simulink model "s_b16a4x512f"  (R2016b)
settings: Solver=VariableStepDiscrete  StartTime=0.0  StopTime=1  RelTol=1e-3
undefined symbols (not defined in the file): fft_stages, n_bits_ants, n_bits_xengs
libraries: xbsIndex_r4 x23057, casper_library_misc x150, xbsReplacements_r4 x9, casper_library_delays x8, xps_library x3
(part 15 of 210)

== system s_b16a4x512f/tvg_control ==
  convert1_{1..8,11..18} (16 alike) : DataTypeConversion  OutDataTypeStr=fixdt('ufix1_En0')  LockScale=on
  convert1_10 : DataTypeConversion  OutDataTypeStr=fixdt('ufix2_En0')  LockScale=on
  convert1_9 : DataTypeConversion  OutDataTypeStr=fixdt('ufix2_En0')  LockScale=on
  convert2_{1..8,11..18} (16 alike) : DataTypeConversion  OutDataTypeStr=fixdt('ufix1_En0')  ConvertRealWorld=Stored Integer (SI)  LockScale=on
  convert2_10 : DataTypeConversion  OutDataTypeStr=fixdt('ufix2_En0')  ConvertRealWorld=Stored Integer (SI)  LockScale=on
  convert2_9 : DataTypeConversion  OutDataTypeStr=fixdt('ufix2_En0')  ConvertRealWorld=Stored Integer (SI)  LockScale=on
  gain_1 : Gain  Gain=524288
  gain_10 : Gain  Gain=256
  gain_11 : Gain  Gain=128
  gain_12 : Gain  Gain=64
  gain_13 : Gain  Gain=32
  gain_14 : Gain  Gain=16
  gain_15 : Gain  Gain=8
  gain_16 : Gain  Gain=4
  gain_17 : Gain  Gain=2
  gain_18 : Gain
  gain_2 : Gain  Gain=262144
  gain_3 : Gain  Gain=131072
  gain_4 : Gain  Gain=65536
  gain_5 : Gain  Gain=32768
  gain_6 : Gain  Gain=16384
  gain_7 : Gain  Gain=8192
  gain_8 : Gain  Gain=4096
  gain_9 : Gain  Gain=1024
  io_delay : xbsIndex_r4/Delay  rst=off  infoeditControl=Selection of Reset will increase slice count due to use of real FFs and instead of SRLs  en=off  latency=0  reg_retiming=on  dbl_ovrd=off  block_type=delay
      settings: infoedit=Hardware notes: A delay line is a chain, each link of which is an SRL16 or SRL32 followed by a flip-flop.
  reint{9..10,17..18} (4 alike) : xbsIndex_r4/Reinterpret  force_arith_type=on  arith_type=Unsigned  force_bin_pt=on  bin_pt=0  block_type=reinterpret
  s_b16a4x512f_tvg_control_user_data_out : xbsIndex_r4/Gateway In  gui_display_data_type=Fixed-point  arith_type=Unsigned  n_bits=32  bin_pt=0  preci_type=Single  exp_width=8  frac_width=24  rows=1  columns=1  quantization="Round  (unbiased: +/- Inf)"  overflow=Saturate  period=1  UseAsADC=off  ADCChannel='1'  interface=None  automatic_assignment=on  address_offset=hex2dec('00')  intf_name=''  intf_description=''  default_value=0  timing_constraint=None  locs_specified=off  LOCs={}  io_standard={}  inherit_from_input=off  hdl_port=on  dbl_ovrd=off  block_type=gatewayin
  sim_{1..18} (18 alike) : Constant  Value=0
  sim_add : Sum  Inputs=++++++++++++++++++  OutDataTypeStr=uint32
  slice_preproc_snap_dv_mux : xbsIndex_r4/Slice  nbits=1  boolean_output=on  mode=Lower Bit Location + Width  bit1=0  base1=MSB of Input  bit0=6  base0=LSB of Input  dbl_ovrd=off  block_type=slice
  slice_preproc_snap_stop_mux : xbsIndex_r4/Slice  nbits=1  boolean_output=off  mode=Lower Bit Location + Width  bit1=0  base1=MSB of Input  bit0=1  base0=LSB of Input  dbl_ovrd=off  block_type=slice
  slice_reord_snap_dv_arm : xbsIndex_r4/Slice  nbits=1  boolean_output=on  mode=Lower Bit Location + Width  bit1=0  base1=MSB of Input  bit0=7  base0=LSB of Input  dbl_ovrd=off  block_type=slice
  slice_reord_snap_dv_mux : xbsIndex_r4/Slice  nbits=2  boolean_output=off  mode=Lower Bit Location + Width  bit1=0  base1=MSB of Input  bit0=10  base0=LSB of Input  dbl_ovrd=off  block_type=slice
  slice_snap_hmc_pkt_mux_we_sel : xbsIndex_r4/Slice  nbits=1  boolean_output=off  mode=Lower Bit Location + Width  bit1=0  base1=MSB of Input  bit0=0  base0=LSB of Input  dbl_ovrd=off  block_type=slice
  slice_snap_reord_stop_sel : xbsIndex_r4/Slice  nbits=1  boolean_output=on  mode=Lower Bit Location + Width  bit1=0  base1=MSB of Input  bit0=5  base0=LSB of Input  dbl_ovrd=off  block_type=slice
  slice_vacc_tvg_ctr_en : xbsIndex_r4/Slice  nbits=1  boolean_output=on  mode=Lower Bit Location + Width  bit1=0  base1=MSB of Input  bit0=14  base0=LSB of Input  dbl_ovrd=off  block_type=slice
  slice_vacc_tvg_data_sel : xbsIndex_r4/Slice  nbits=1  boolean_output=on  mode=Lower Bit Location + Width  bit1=0  base1=MSB of Input  bit0=16  base0=LSB of Input  dbl_ovrd=off  block_type=slice
  slice_vacc_tvg_pulse_en : xbsIndex_r4/Slice  nbits=1  boolean_output=on  mode=Lower Bit Location + Width  bit1=0  base1=MSB of Input  bit0=19  base0=LSB of Input  dbl_ovrd=off  block_type=slice
  slice_vacc_tvg_reset : xbsIndex_r4/Slice  nbits=1  boolean_output=on  mode=Lower Bit Location + Width  bit1=0  base1=MSB of Input  bit0=15  base0=LSB of Input  dbl_ovrd=off  block_type=slice
  slice_vacc_tvg_run : xbsIndex_r4/Slice  nbits=1  boolean_output=on  mode=Lower Bit Location + Width  bit1=0  base1=MSB of Input  bit0=12  base0=LSB of Input  dbl_ovrd=off  block_type=slice
  slice_vacc_tvg_sync_sel : xbsIndex_r4/Slice  nbits=1  boolean_output=on  mode=Lower Bit Location + Width  bit1=0  base1=MSB of Input  bit0=18  base0=LSB of Input  dbl_ovrd=off  block_type=slice
  slice_vacc_tvg_valid_sel : xbsIndex_r4/Slice  nbits=1  boolean_output=on  mode=Lower Bit Location + Width  bit1=0  base1=MSB of Input  bit0=17  base0=LSB of Input  dbl_ovrd=off  block_type=slice
  slice_vacc_tvg_vector_en : xbsIndex_r4/Slice  nbits=1  boolean_output=on  mode=Lower Bit Location + Width  bit1=0  base1=MSB of Input  bit0=13  base0=LSB of Input  dbl_ovrd=off  block_type=slice
  slice_xeng_tvg_data_sel : xbsIndex_r4/Slice  nbits=2  boolean_output=off  mode=Lower Bit Location + Width  bit1=0  base1=MSB of Input  bit0=8  base0=LSB of Input  dbl_ovrd=off  block_type=slice
  slice_xeng_tvg_inj_vector : xbsIndex_r4/Slice  nbits=1  boolean_output=on  mode=Lower Bit Location + Width  bit1=0  base1=MSB of Input  bit0=3  base0=LSB of Input  dbl_ovrd=off  block_type=slice
  slice_xeng_tvg_mcnt_sel : xbsIndex_r4/Slice  nbits=1  boolean_output=on  mode=Lower Bit Location + Width  bit1=0  base1=MSB of Input  bit0=2  base0=LSB of Input  dbl_ovrd=off  block_type=slice
  slice_xeng_tvg_val_sel : xbsIndex_r4/Slice  nbits=1  boolean_output=on  mode=Lower Bit Location + Width  bit1=0  base1=MSB of Input  bit0=4  base0=LSB of Input  dbl_ovrd=off  block_type=slice
  in_vacc_tvg_pulse_en : Outport
  in_vacc_tvg_sync_sel : Outport  Port=2
  in_vacc_tvg_valid_sel : Outport  Port=3
  in_vacc_tvg_data_sel : Outport  Port=4
  in_vacc_tvg_reset : Outport  Port=5
  in_vacc_tvg_ctr_en : Outport  Port=6
  in_vacc_tvg_vector_en : Outport  Port=7
  in_vacc_tvg_run : Outport  Port=8
  in_reord_snap_dv_mux : Outport  Port=9
  in_xeng_tvg_data_sel : Outport  Port=10
  in_reord_snap_dv_arm : Outport  Port=11
  in_preproc_snap_dv_mux : Outport  Port=12
  in_snap_reord_stop_sel : Outport  Port=13
  in_xeng_tvg_val_sel : Outport  Port=14
  in_xeng_tvg_inj_vector : Outport  Port=15
  in_xeng_tvg_mcnt_sel : Outport  Port=16
  in_preproc_snap_stop_mux : Outport  Port=17
  in_snap_hmc_pkt_mux_we_sel : Outport  Port=18
  wires:
  s_b16a4x512f_tvg_control_user_data_out/1 -> io_delay/1
  sim_add/1 -> s_b16a4x512f_tvg_control_user_data_out/1
  sim_1/1 -> convert1_1/1
  convert1_1/1 -> convert2_1/1
  convert2_1/1 -> gain_1/1
  gain_1/1 -> sim_add/1
  io_delay/1 -> slice_vacc_tvg_pulse_en/1, slice_vacc_tvg_sync_sel/1, slice_vacc_tvg_valid_sel/1, slice_vacc_tvg_data_sel/1, slice_vacc_tvg_reset/1, slice_vacc_tvg_ctr_en/1, slice_vacc_tvg_vector_en/1, slice_vacc_tvg_run/1, slice_reord_snap_dv_mux/1, slice_xeng_tvg_data_sel/1, slice_reord_snap_dv_arm/1, slice_preproc_snap_dv_mux/1, slice_snap_reord_stop_sel/1, slice_xeng_tvg_val_sel/1, slice_xeng_tvg_inj_vector/1, slice_xeng_tvg_mcnt_sel/1, slice_preproc_snap_stop_mux/1, slice_snap_hmc_pkt_mux_we_sel/1
  slice_vacc_tvg_pulse_en/1 -> in_vacc_tvg_pulse_en/1
  sim_2/1 -> convert1_2/1
  convert1_2/1 -> convert2_2/1
  convert2_2/1 -> gain_2/1
  gain_2/1 -> sim_add/2
  slice_vacc_tvg_sync_sel/1 -> in_vacc_tvg_sync_sel/1
  sim_3/1 -> convert1_3/1
  convert1_3/1 -> convert2_3/1
  convert2_3/1 -> gain_3/1
  gain_3/1 -> sim_add/3
  slice_vacc_tvg_valid_sel/1 -> in_vacc_tvg_valid_sel/1
  sim_4/1 -> convert1_4/1
  convert1_4/1 -> convert2_4/1
  convert2_4/1 -> gain_4/1
  gain_4/1 -> sim_add/4
  slice_vacc_tvg_data_sel/1 -> in_vacc_tvg_data_sel/1
  sim_5/1 -> convert1_5/1
  convert1_5/1 -> convert2_5/1
  convert2_5/1 -> gain_5/1
  gain_5/1 -> sim_add/5
  slice_vacc_tvg_reset/1 -> in_vacc_tvg_reset/1
  sim_6/1 -> convert1_6/1
  convert1_6/1 -> convert2_6/1
  convert2_6/1 -> gain_6/1
  gain_6/1 -> sim_add/6
  slice_vacc_tvg_ctr_en/1 -> in_vacc_tvg_ctr_en/1
  sim_7/1 -> convert1_7/1
  convert1_7/1 -> convert2_7/1
  convert2_7/1 -> gain_7/1
  gain_7/1 -> sim_add/7
  slice_vacc_tvg_vector_en/1 -> in_vacc_tvg_vector_en/1
  sim_8/1 -> convert1_8/1
  convert1_8/1 -> convert2_8/1
  convert2_8/1 -> gain_8/1
  gain_8/1 -> sim_add/8
  slice_vacc_tvg_run/1 -> in_vacc_tvg_run/1
  sim_9/1 -> convert1_9/1
  convert1_9/1 -> convert2_9/1
  convert2_9/1 -> gain_9/1
  gain_9/1 -> sim_add/9
  slice_reord_snap_dv_mux/1 -> reint9/1
  reint9/1 -> in_reord_snap_dv_mux/1
  sim_10/1 -> convert1_10/1
  convert1_10/1 -> convert2_10/1
  convert2_10/1 -> gain_10/1
  gain_10/1 -> sim_add/10
  slice_xeng_tvg_data_sel/1 -> reint10/1
  reint10/1 -> in_xeng_tvg_data_sel/1
  sim_11/1 -> convert1_11/1
  convert1_11/1 -> convert2_11/1
  convert2_11/1 -> gain_11/1
  gain_11/1 -> sim_add/11
  slice_reord_snap_dv_arm/1 -> in_reord_snap_dv_arm/1
  sim_12/1 -> convert1_12/1
  convert1_12/1 -> convert2_12/1
  convert2_12/1 -> gain_12/1
  gain_12/1 -> sim_add/12
  slice_preproc_snap_dv_mux/1 -> in_preproc_snap_dv_mux/1
  sim_13/1 -> convert1_13/1
  convert1_13/1 -> convert2_13/1
  convert2_13/1 -> gain_13/1
  gain_13/1 -> sim_add/13
  slice_snap_reord_stop_sel/1 -> in_snap_reord_stop_sel/1
  sim_14/1 -> convert1_14/1
  convert1_14/1 -> convert2_14/1
  convert2_14/1 -> gain_14/1
  gain_14/1 -> sim_add/14
  slice_xeng_tvg_val_sel/1 -> in_xeng_tvg_val_sel/1
  sim_15/1 -> convert1_15/1
  convert1_15/1 -> convert2_15/1
  convert2_15/1 -> gain_15/1
  gain_15/1 -> sim_add/15
  slice_xeng_tvg_inj_vector/1 -> in_xeng_tvg_inj_vector/1
  sim_16/1 -> convert1_16/1
  convert1_16/1 -> convert2_16/1
  convert2_16/1 -> gain_16/1
  gain_16/1 -> sim_add/16
  slice_xeng_tvg_mcnt_sel/1 -> in_xeng_tvg_mcnt_sel/1
  sim_17/1 -> convert1_17/1
  convert1_17/1 -> convert2_17/1
  convert2_17/1 -> gain_17/1
  gain_17/1 -> sim_add/17
  slice_preproc_snap_stop_mux/1 -> reint17/1
  reint17/1 -> in_preproc_snap_stop_mux/1
  sim_18/1 -> convert1_18/1
  convert1_18/1 -> convert2_18/1
  convert2_18/1 -> gain_18/1
  gain_18/1 -> sim_add/18
  slice_snap_hmc_pkt_mux_we_sel/1 -> reint18/1
  reint18/1 -> in_snap_hmc_pkt_mux_we_sel/1

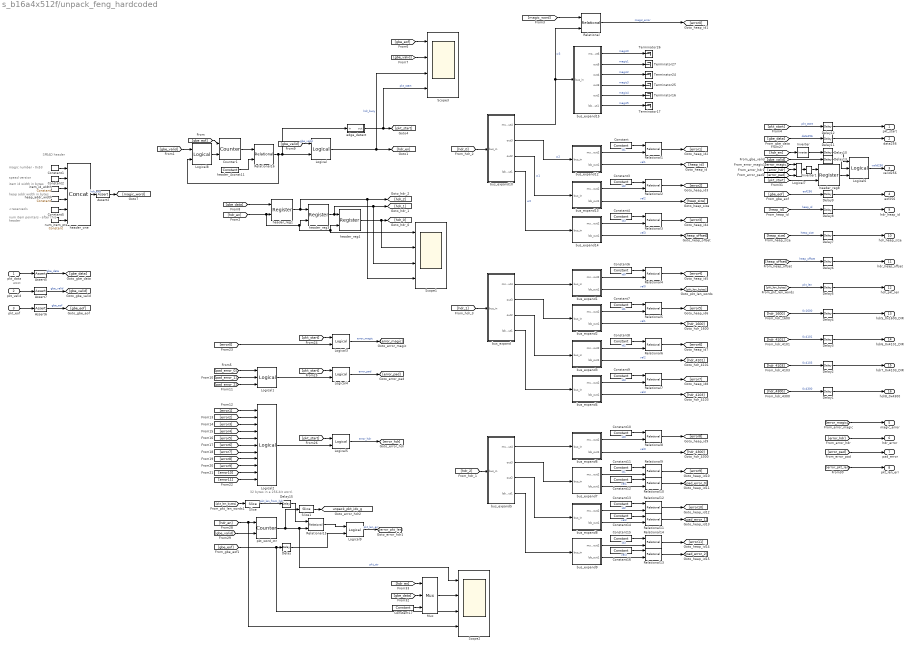
== system s_b16a4x512f/unpack_feng_hardcoded ==
  note: 32 bytes in a 256-bit word.
  note: woot
  note: SPEAD header
  note: magic number - 0x53
  note: spead version
  note: item id width in bytes
  note: heap addr width in bytes
  note: <reserved>
  note: num item pointers -
      | after this header
  pkt_data : Inport
  pkt_valid : Inport  Port=2
  pkt_eof : Inport  Port=3
  Assert2 : xbsIndex_r4/Assert  assert_type=on  type_source=Explicitly  gui_display_data_type=Fixed-point  arith_type=Unsigned  n_bits=64  bin_pt=0  preci_type=Single  exp_width=8  frac_width=24  assert_rate=off  rate_source=Explicitly  period=1  output_port=on  block_type=assert
      settings: block_version=10.1.3
  Assert5 : xbsIndex_r4/Assert  assert_type=on  type_source=Explicitly  gui_display_data_type=Fixed-point  arith_type=Unsigned  n_bits=256  bin_pt=0  preci_type=Single  exp_width=8  frac_width=24  assert_rate=off  rate_source=Explicitly  period=1  output_port=on  block_type=assert
      settings: block_version=10.1.3
  Assert6 : xbsIndex_r4/Assert  assert_type=on  type_source=Explicitly  gui_display_data_type=Boolean  arith_type=Boolean  n_bits=spead_msw  bin_pt=0  preci_type=Single  exp_width=8  frac_width=24  assert_rate=off  rate_source=Explicitly  period=1  output_port=on  block_type=assert
      settings: block_version=10.1.3
  Assert7 : xbsIndex_r4/Assert  assert_type=on  type_source=Explicitly  gui_display_data_type=Boolean  arith_type=Boolean  n_bits=64  bin_pt=0  preci_type=Single  exp_width=8  frac_width=24  assert_rate=off  rate_source=Explicitly  period=1  output_port=on  block_type=assert
      settings: block_version=10.1.3
  Constant : xbsIndex_r4/Constant  const=32769  gui_display_data_type=Fixed-point  arith_type=Unsigned  n_bits=16  bin_pt=0  preci_type=Single  exp_width=8  frac_width=24  explicit_period=on  period=1  equ=P=C  opselect=C  inp2=PCIN>>17  opr=+  inp1=P  carry=CIN  dbl_ovrd=off  block_type=constant
  Constant1 : xbsIndex_r4/Constant  const=83  gui_display_data_type=Fixed-point  arith_type=Unsigned  n_bits=8  bin_pt=0  preci_type=Single  exp_width=8  frac_width=24  explicit_period=on  period=1  equ=P=C  opselect=C  inp2=PCIN>>17  opr=+  inp1=P  carry=CIN  dbl_ovrd=off  block_type=constant
  Constant10 : xbsIndex_r4/Constant  const=hex2dec('4300')  gui_display_data_type=Fixed-point  arith_type=Unsigned  n_bits=16  bin_pt=0  preci_type=Single  exp_width=8  frac_width=24  explicit_period=on  period=1  equ=P=C  opselect=C  inp2=PCIN>>17  opr=+  inp1=P  carry=CIN  dbl_ovrd=off  block_type=constant
  Constant11 : xbsIndex_r4/Constant  const=2^15  gui_display_data_type=Fixed-point  arith_type=Unsigned  n_bits=16  bin_pt=0  preci_type=Single  exp_width=8  frac_width=24  explicit_period=on  period=1  equ=P=C  opselect=C  inp2=PCIN>>17  opr=+  inp1=P  carry=CIN  dbl_ovrd=off  block_type=constant
  Constant12 : xbsIndex_r4/Constant  const=0  gui_display_data_type=Fixed-point  arith_type=Unsigned  n_bits=48  bin_pt=0  preci_type=Single  exp_width=8  frac_width=24  explicit_period=on  period=1  equ=P=C  opselect=C  inp2=PCIN>>17  opr=+  inp1=P  carry=CIN  dbl_ovrd=off  block_type=constant
  Constant13 : xbsIndex_r4/Constant  const=2^15  gui_display_data_type=Fixed-point  arith_type=Unsigned  n_bits=16  bin_pt=0  preci_type=Single  exp_width=8  frac_width=24  explicit_period=on  period=1  equ=P=C  opselect=C  inp2=PCIN>>17  opr=+  inp1=P  carry=CIN  dbl_ovrd=off  block_type=constant
  Constant14 : xbsIndex_r4/Constant  const=0  gui_display_data_type=Fixed-point  arith_type=Unsigned  n_bits=48  bin_pt=0  preci_type=Single  exp_width=8  frac_width=24  explicit_period=on  period=1  equ=P=C  opselect=C  inp2=PCIN>>17  opr=+  inp1=P  carry=CIN  dbl_ovrd=off  block_type=constant
  Constant15 : xbsIndex_r4/Constant  const=2^15  gui_display_data_type=Fixed-point  arith_type=Unsigned  n_bits=16  bin_pt=0  preci_type=Single  exp_width=8  frac_width=24  explicit_period=on  period=1  equ=P=C  opselect=C  inp2=PCIN>>17  opr=+  inp1=P  carry=CIN  dbl_ovrd=off  block_type=constant
  Constant16 : xbsIndex_r4/Constant  const=0  gui_display_data_type=Fixed-point  arith_type=Unsigned  n_bits=48  bin_pt=0  preci_type=Single  exp_width=8  frac_width=24  explicit_period=on  period=1  equ=P=C  opselect=C  inp2=PCIN>>17  opr=+  inp1=P  carry=CIN  dbl_ovrd=off  block_type=constant
  Constant17 : xbsIndex_r4/Constant  const=0  gui_display_data_type=Fixed-point  arith_type=Unsigned  n_bits=256  bin_pt=0  preci_type=Single  exp_width=8  frac_width=24  explicit_period=on  period=1  equ=P=C  opselect=C  inp2=PCIN>>17  opr=+  inp1=P  carry=CIN  dbl_ovrd=off  block_type=constant
  Constant2 : xbsIndex_r4/Constant  const=spead_version  gui_display_data_type=Fixed-point  arith_type=Unsigned  n_bits=8  bin_pt=0  preci_type=Single  exp_width=8  frac_width=24  explicit_period=on  period=1  equ=P=C  opselect=C  inp2=PCIN>>17  opr=+  inp1=P  carry=CIN  dbl_ovrd=off  block_type=constant
  Constant3 : xbsIndex_r4/Constant  const=32770  gui_display_data_type=Fixed-point  arith_type=Unsigned  n_bits=16  bin_pt=0  preci_type=Single  exp_width=8  frac_width=24  explicit_period=on  period=1  equ=P=C  opselect=C  inp2=PCIN>>17  opr=+  inp1=P  carry=CIN  dbl_ovrd=off  block_type=constant
  Constant4 : xbsIndex_r4/Constant  const=32771  gui_display_data_type=Fixed-point  arith_type=Unsigned  n_bits=16  bin_pt=0  preci_type=Single  exp_width=8  frac_width=24  explicit_period=on  period=1  equ=P=C  opselect=C  inp2=PCIN>>17  opr=+  inp1=P  carry=CIN  dbl_ovrd=off  block_type=constant
  Constant5 : xbsIndex_r4/Constant  const=0  gui_display_data_type=Fixed-point  arith_type=Unsigned  n_bits=16  bin_pt=0  preci_type=Single  exp_width=8  frac_width=24  explicit_period=on  period=1  equ=P=C  opselect=C  inp2=PCIN>>17  opr=+  inp1=P  carry=CIN  dbl_ovrd=off  block_type=constant
  Constant6 : xbsIndex_r4/Constant  const=32772  gui_display_data_type=Fixed-point  arith_type=Unsigned  n_bits=16  bin_pt=0  preci_type=Single  exp_width=8  frac_width=24  explicit_period=on  period=1  equ=P=C  opselect=C  inp2=PCIN>>17  opr=+  inp1=P  carry=CIN  dbl_ovrd=off  block_type=constant
  Constant7 : xbsIndex_r4/Constant  const=hex2dec('1600') + pow2(15)  gui_display_data_type=Fixed-point  arith_type=Unsigned  n_bits=16  bin_pt=0  preci_type=Single  exp_width=8  frac_width=24  explicit_period=on  period=1  equ=P=C  opselect=C  inp2=PCIN>>17  opr=+  inp1=P  carry=CIN  dbl_ovrd=off  block_type=constant
  Constant8 : xbsIndex_r4/Constant  const=hex2dec('4101') + pow2(15)  gui_display_data_type=Fixed-point  arith_type=Unsigned  n_bits=16  bin_pt=0  preci_type=Single  exp_width=8  frac_width=24  explicit_period=on  period=1  equ=P=C  opselect=C  inp2=PCIN>>17  opr=+  inp1=P  carry=CIN  dbl_ovrd=off  block_type=constant
  Constant9 : xbsIndex_r4/Constant  const=hex2dec('4103') + pow2(15)  gui_display_data_type=Fixed-point  arith_type=Unsigned  n_bits=16  bin_pt=0  preci_type=Single  exp_width=8  frac_width=24  explicit_period=on  period=1  equ=P=C  opselect=C  inp2=PCIN>>17  opr=+  inp1=P  carry=CIN  dbl_ovrd=off  block_type=constant
  Counter1 : xbsIndex_r4/Counter  cnt_type=Free Running  cnt_to=1  operation=Up  start_count=0  cnt_by_val=1  arith_type=Unsigned  n_bits=max_pkt_len_bits-2  bin_pt=0  load_pin=off  rst=on  en=on  explicit_period=on  period=1  use_behavioral_HDL=off  implementation=Fabric  dbl_ovrd=off  block_type=counter
  Delay{,1..13,15} (15 alike) : xbsIndex_r4/Delay  rst=off  infoeditControl=Selection of Reset will increase slice count due to use of real FFs and instead of SRLs  en=off  latency=1  reg_retiming=off  dbl_ovrd=off  block_type=delay
      settings: infoedit=Hardware notes: A delay line is a chain, each link of which is an SRL16 or SRL32 followed by a flip-flop.
  Inverter : xbsIndex_r4/Inverter  en=off  latency=0  dbl_ovrd=off  block_type=inv
  Inverter1 : xbsIndex_r4/Inverter  en=off  latency=0  dbl_ovrd=off  block_type=inv
  Logical{,3..5,8..9} (6 alike) : xbsIndex_r4/Logical  logical_function=AND  inputs=2  en=off  latency=0  precision=Full  arith_type=Unsigned  n_bits=16  bin_pt=0  align_bp=on  dbl_ovrd=off  block_type=logical
  Logical1 : xbsIndex_r4/Logical  logical_function=OR  inputs=3  en=off  latency=0  precision=Full  arith_type=Unsigned  n_bits=16  bin_pt=0  align_bp=on  dbl_ovrd=off  block_type=logical
  Logical2 : xbsIndex_r4/Logical  logical_function=OR  inputs=11  en=off  latency=0  precision=Full  arith_type=Unsigned  n_bits=16  bin_pt=0  align_bp=on  dbl_ovrd=off  block_type=logical
  Logical6 : xbsIndex_r4/Logical  logical_function=AND  inputs=3  en=off  latency=0  precision=Full  arith_type=Unsigned  n_bits=16  bin_pt=0  align_bp=on  dbl_ovrd=off  block_type=logical
  Logical7 : xbsIndex_r4/Logical  logical_function=OR  inputs=3  en=off  latency=0  precision=Full  arith_type=Unsigned  n_bits=16  bin_pt=0  align_bp=on  dbl_ovrd=off  block_type=logical
  Mux : xbsIndex_r4/Mux  inputs=2  en=off  latency=0  precision=Full  arith_type=Unsigned  n_bits=16  bin_pt=14  quantization=Truncate  overflow=Wrap  dbl_ovrd=off  block_type=mux
  Relational{,1..15} (16 alike) : xbsIndex_r4/Relational  mode=a!=b  op_type=Bool  en=off  latency=0  dbl_ovrd=off  block_type=relational
  Relational16 : xbsIndex_r4/Relational  mode=a<=b  op_type=Bool  en=off  latency=0  dbl_ovrd=off  block_type=relational
  Scope1 : Scope  NumInputPorts=4
  Scope2 : Scope  NumInputPorts=4
  Scope3 : Scope  NumInputPorts=4
  Slice : xbsIndex_r4/Slice  nbits=max_pkt_len_bits-2  boolean_output=off  mode=Lower Bit Location + Width  bit1=0  base1=MSB of Input  bit0=5  base0=LSB of Input  dbl_ovrd=off  block_type=slice
  Slice1 : xbsIndex_r4/Slice  nbits=5  boolean_output=off  mode=Lower Bit Location + Width  bit1=0  base1=MSB of Input  bit0=0  base0=LSB of Input  dbl_ovrd=off  block_type=slice
  Terminator{16..17,24..27} (6 alike) : Terminator
  bus_expand : Subsystem  AncestorBlock=casper_library_flow_control/bus_expand  mask(bus_expand){mode=divisions of equal size, outputNum=4, outputWidth=64, outputBinaryPt=0, outputArithmeticType=0, show_format=on, outputToWorkspace=off, variablePrefix=out, outputToModelAsWell=on}
      mask prompts: outputNum "Number of outputs:"; outputWidth "Output width:"; outputBinaryPt "Output binary point position:"; outputArithmeticType "Output arithmetic type (ufix=0, fix=1, bool=2):"; show_format "Print format string?"; outputToWorkspace "Output to workspace?"; variablePrefix "Variable name prefix:"; outputToModelAsWell "Output to model as well?"
      mask help:
      | Expands a 'bus' made using a bus_create or Xilinx
      | concat block.
      | The input will be divided into the specified number
      | of outputs with the specified arithmetic types.
      | Divisions are made from most significant bit.
      mask init: same as s_b16a4x512f/bus_expand
      settings: AttributesFormatString=4 outputs: uf64.0,uf64.0,uf64.0,uf64.0,
      mask TypeOptions mode: divisions of equal size | divisions of arbitrary size
      mask Callback mode: bus_expand_callback();
      mask Callback outputWidth: bus_expand_callback();
      mask Callback outputToWorkspace: bus_expand_callback();
  bus_expand1 : Subsystem  AncestorBlock=casper_library_flow_control/bus_expand  mask(bus_expand){mode=divisions of arbitrary size, outputNum=1, outputWidth=[16 48], outputBinaryPt=0, outputArithmeticType=0, show_format=on, outputToWorkspace=off, variablePrefix=out, outputToModelAsWell=on}
      mask prompts: outputNum "Number of outputs:"; outputWidth "Output width [msb ... lsb]:"; outputBinaryPt "Output binary point position [msb ... lsb]:"; outputArithmeticType "Output arithmetic type (ufix=0, fix=1, bool=2) [msb ... lsb]:"; show_format "Print format string?"; outputToWorkspace "Output to workspace?"; variablePrefix "Variable name prefix:"; outputToModelAsWell "Output to model as well?"
      mask help:
      | Expands a 'bus' made using a bus_create or Xilinx
      | concat block.
      | The input will be divided into the specified number
      | of outputs with the specified arithmetic types.
      | Divisions are made from most significant bit.
      mask init: same as s_b16a4x512f/bus_expand
      settings: AttributesFormatString=2 outputs: uf16.0,uf48.0,
      mask TypeOptions mode: divisions of equal size | divisions of arbitrary size
      mask Callback mode: bus_expand_callback();
      mask Callback outputWidth: bus_expand_callback();
      mask Callback outputToWorkspace: bus_expand_callback();
  bus_expand10 : Subsystem  AncestorBlock=casper_library_flow_control/bus_expand  mask(bus_expand){mode=divisions of equal size, outputNum=4, outputWidth=64, outputBinaryPt=0, outputArithmeticType=0, show_format=on, outputToWorkspace=off, variablePrefix=out, outputToModelAsWell=on}
      mask prompts: outputNum "Number of outputs:"; outputWidth "Output width:"; outputBinaryPt "Output binary point position:"; outputArithmeticType "Output arithmetic type (ufix=0, fix=1, bool=2):"; show_format "Print format string?"; outputToWorkspace "Output to workspace?"; variablePrefix "Variable name prefix:"; outputToModelAsWell "Output to model as well?"
      mask help:
      | Expands a 'bus' made using a bus_create or Xilinx
      | concat block.
      | The input will be divided into the specified number
      | of outputs with the specified arithmetic types.
      | Divisions are made from most significant bit.
      mask init: same as s_b16a4x512f/bus_expand
      settings: AttributesFormatString=4 outputs: uf64.0,uf64.0,uf64.0,uf64.0,
      mask TypeOptions mode: divisions of equal size | divisions of arbitrary size
      mask Callback mode: bus_expand_callback();
      mask Callback outputWidth: bus_expand_callback();
      mask Callback outputToWorkspace: bus_expand_callback();
  bus_expand12 : Subsystem  AncestorBlock=casper_library_flow_control/bus_expand  mask(bus_expand){mode=divisions of arbitrary size, outputNum=1, outputWidth=[16 48], outputBinaryPt=0, outputArithmeticType=0, show_format=on, outputToWorkspace=off, variablePrefix=out, outputToModelAsWell=on}
      mask prompts: outputNum "Number of outputs:"; outputWidth "Output width [msb ... lsb]:"; outputBinaryPt "Output binary point position [msb ... lsb]:"; outputArithmeticType "Output arithmetic type (ufix=0, fix=1, bool=2) [msb ... lsb]:"; show_format "Print format string?"; outputToWorkspace "Output to workspace?"; variablePrefix "Variable name prefix:"; outputToModelAsWell "Output to model as well?"
      mask help:
      | Expands a 'bus' made using a bus_create or Xilinx
      | concat block.
      | The input will be divided into the specified number
      | of outputs with the specified arithmetic types.
      | Divisions are made from most significant bit.
      mask init: same as s_b16a4x512f/bus_expand
      settings: AttributesFormatString=2 outputs: uf16.0,uf48.0,
      mask TypeOptions mode: divisions of equal size | divisions of arbitrary size
      mask Callback mode: bus_expand_callback();
      mask Callback outputWidth: bus_expand_callback();
      mask Callback outputToWorkspace: bus_expand_callback();
  bus_expand13 : Subsystem  AncestorBlock=casper_library_flow_control/bus_expand  mask(bus_expand){mode=divisions of arbitrary size, outputNum=1, outputWidth=[16 48], outputBinaryPt=0, outputArithmeticType=0, show_format=on, outputToWorkspace=off, variablePrefix=out, outputToModelAsWell=on}
      mask prompts: outputNum "Number of outputs:"; outputWidth "Output width [msb ... lsb]:"; outputBinaryPt "Output binary point position [msb ... lsb]:"; outputArithmeticType "Output arithmetic type (ufix=0, fix=1, bool=2) [msb ... lsb]:"; show_format "Print format string?"; outputToWorkspace "Output to workspace?"; variablePrefix "Variable name prefix:"; outputToModelAsWell "Output to model as well?"
      mask help:
      | Expands a 'bus' made using a bus_create or Xilinx
      | concat block.
      | The input will be divided into the specified number
      | of outputs with the specified arithmetic types.
      | Divisions are made from most significant bit.
      mask init: same as s_b16a4x512f/bus_expand
      settings: AttributesFormatString=2 outputs: uf16.0,uf48.0,
      mask TypeOptions mode: divisions of equal size | divisions of arbitrary size
      mask Callback mode: bus_expand_callback();
      mask Callback outputWidth: bus_expand_callback();
      mask Callback outputToWorkspace: bus_expand_callback();
  bus_expand14 : Subsystem  AncestorBlock=casper_library_flow_control/bus_expand  mask(bus_expand){mode=divisions of arbitrary size, outputNum=1, outputWidth=[16 48], outputBinaryPt=0, outputArithmeticType=0, show_format=on, outputToWorkspace=off, variablePrefix=out, outputToModelAsWell=on}
      mask prompts: outputNum "Number of outputs:"; outputWidth "Output width [msb ... lsb]:"; outputBinaryPt "Output binary point position [msb ... lsb]:"; outputArithmeticType "Output arithmetic type (ufix=0, fix=1, bool=2) [msb ... lsb]:"; show_format "Print format string?"; outputToWorkspace "Output to workspace?"; variablePrefix "Variable name prefix:"; outputToModelAsWell "Output to model as well?"
      mask help:
      | Expands a 'bus' made using a bus_create or Xilinx
      | concat block.
      | The input will be divided into the specified number
      | of outputs with the specified arithmetic types.
      | Divisions are made from most significant bit.
      mask init: same as s_b16a4x512f/bus_expand
      settings: AttributesFormatString=2 outputs: uf16.0,uf48.0,
      mask TypeOptions mode: divisions of equal size | divisions of arbitrary size
      mask Callback mode: bus_expand_callback();
      mask Callback outputWidth: bus_expand_callback();
      mask Callback outputToWorkspace: bus_expand_callback();
  bus_expand15 : Subsystem  AncestorBlock=casper_library_flow_control/bus_expand  mask(bus_expand){mode=divisions of arbitrary size, outputNum=1, outputWidth=[8 8 8 8 16 16], outputBinaryPt=0, outputArithmeticType=0, show_format=on, outputToWorkspace=off, variablePrefix=out, outputToModelAsWell=on}
      mask prompts: outputNum "Number of outputs:"; outputWidth "Output width [msb ... lsb]:"; outputBinaryPt "Output binary point position [msb ... lsb]:"; outputArithmeticType "Output arithmetic type (ufix=0, fix=1, bool=2) [msb ... lsb]:"; show_format "Print format string?"; outputToWorkspace "Output to workspace?"; variablePrefix "Variable name prefix:"; outputToModelAsWell "Output to model as well?"
      mask help:
      | Expands a 'bus' made using a bus_create or Xilinx
      | concat block.
      | The input will be divided into the specified number
      | of outputs with the specified arithmetic types.
      | Divisions are made from most significant bit.
      mask init: same as s_b16a4x512f/bus_expand
      settings: AttributesFormatString=6 outputs: uf8.0,uf8.0,uf8.0,uf8.0,uf16.0,uf16.0,
      mask TypeOptions mode: divisions of equal size | divisions of arbitrary size
      mask Callback mode: bus_expand_callback();
      mask Callback outputWidth: bus_expand_callback();
      mask Callback outputToWorkspace: bus_expand_callback();
  bus_expand2 : Subsystem  AncestorBlock=casper_library_flow_control/bus_expand  mask(bus_expand){mode=divisions of arbitrary size, outputNum=1, outputWidth=[16 48], outputBinaryPt=0, outputArithmeticType=0, show_format=on, outputToWorkspace=off, variablePrefix=out, outputToModelAsWell=on}
      mask prompts: outputNum "Number of outputs:"; outputWidth "Output width [msb ... lsb]:"; outputBinaryPt "Output binary point position [msb ... lsb]:"; outputArithmeticType "Output arithmetic type (ufix=0, fix=1, bool=2) [msb ... lsb]:"; show_format "Print format string?"; outputToWorkspace "Output to workspace?"; variablePrefix "Variable name prefix:"; outputToModelAsWell "Output to model as well?"
      mask help:
      | Expands a 'bus' made using a bus_create or Xilinx
      | concat block.
      | The input will be divided into the specified number
      | of outputs with the specified arithmetic types.
      | Divisions are made from most significant bit.
      mask init: same as s_b16a4x512f/bus_expand
      settings: AttributesFormatString=2 outputs: uf16.0,uf48.0,
      mask TypeOptions mode: divisions of equal size | divisions of arbitrary size
      mask Callback mode: bus_expand_callback();
      mask Callback outputWidth: bus_expand_callback();
      mask Callback outputToWorkspace: bus_expand_callback();
  bus_expand3 : Subsystem  AncestorBlock=casper_library_flow_control/bus_expand  mask(bus_expand){mode=divisions of arbitrary size, outputNum=1, outputWidth=[16 48], outputBinaryPt=0, outputArithmeticType=0, show_format=on, outputToWorkspace=off, variablePrefix=out, outputToModelAsWell=on}
      mask prompts: outputNum "Number of outputs:"; outputWidth "Output width [msb ... lsb]:"; outputBinaryPt "Output binary point position [msb ... lsb]:"; outputArithmeticType "Output arithmetic type (ufix=0, fix=1, bool=2) [msb ... lsb]:"; show_format "Print format string?"; outputToWorkspace "Output to workspace?"; variablePrefix "Variable name prefix:"; outputToModelAsWell "Output to model as well?"
      mask help:
      | Expands a 'bus' made using a bus_create or Xilinx
      | concat block.
      | The input will be divided into the specified number
      | of outputs with the specified arithmetic types.
      | Divisions are made from most significant bit.
      mask init: same as s_b16a4x512f/bus_expand
      settings: AttributesFormatString=2 outputs: uf16.0,uf48.0,
      mask TypeOptions mode: divisions of equal size | divisions of arbitrary size
      mask Callback mode: bus_expand_callback();
      mask Callback outputWidth: bus_expand_callback();
      mask Callback outputToWorkspace: bus_expand_callback();
  bus_expand4 : Subsystem  AncestorBlock=casper_library_flow_control/bus_expand  mask(bus_expand){mode=divisions of arbitrary size, outputNum=1, outputWidth=[16 48], outputBinaryPt=0, outputArithmeticType=0, show_format=on, outputToWorkspace=off, variablePrefix=out, outputToModelAsWell=on}
      mask prompts: outputNum "Number of outputs:"; outputWidth "Output width [msb ... lsb]:"; outputBinaryPt "Output binary point position [msb ... lsb]:"; outputArithmeticType "Output arithmetic type (ufix=0, fix=1, bool=2) [msb ... lsb]:"; show_format "Print format string?"; outputToWorkspace "Output to workspace?"; variablePrefix "Variable name prefix:"; outputToModelAsWell "Output to model as well?"
      mask help:
      | Expands a 'bus' made using a bus_create or Xilinx
      | concat block.
      | The input will be divided into the specified number
      | of outputs with the specified arithmetic types.
      | Divisions are made from most significant bit.
      mask init: same as s_b16a4x512f/bus_expand
      settings: AttributesFormatString=2 outputs: uf16.0,uf48.0,
      mask TypeOptions mode: divisions of equal size | divisions of arbitrary size
      mask Callback mode: bus_expand_callback();
      mask Callback outputWidth: bus_expand_callback();
      mask Callback outputToWorkspace: bus_expand_callback();
  bus_expand5 : Subsystem  AncestorBlock=casper_library_flow_control/bus_expand  mask(bus_expand){mode=divisions of equal size, outputNum=4, outputWidth=64, outputBinaryPt=0, outputArithmeticType=0, show_format=on, outputToWorkspace=off, variablePrefix=out, outputToModelAsWell=on}
      mask prompts: outputNum "Number of outputs:"; outputWidth "Output width:"; outputBinaryPt "Output binary point position:"; outputArithmeticType "Output arithmetic type (ufix=0, fix=1, bool=2):"; show_format "Print format string?"; outputToWorkspace "Output to workspace?"; variablePrefix "Variable name prefix:"; outputToModelAsWell "Output to model as well?"
      mask help:
      | Expands a 'bus' made using a bus_create or Xilinx
      | concat block.
      | The input will be divided into the specified number
      | of outputs with the specified arithmetic types.
      | Divisions are made from most significant bit.
      mask init: same as s_b16a4x512f/bus_expand
      settings: AttributesFormatString=4 outputs: uf64.0,uf64.0,uf64.0,uf64.0,
      mask TypeOptions mode: divisions of equal size | divisions of arbitrary size
      mask Callback mode: bus_expand_callback();
      mask Callback outputWidth: bus_expand_callback();
      mask Callback outputToWorkspace: bus_expand_callback();
  bus_expand6 : Subsystem  AncestorBlock=casper_library_flow_control/bus_expand  mask(bus_expand){mode=divisions of arbitrary size, outputNum=1, outputWidth=[16 48], outputBinaryPt=0, outputArithmeticType=0, show_format=on, outputToWorkspace=off, variablePrefix=out, outputToModelAsWell=on}
      mask prompts: outputNum "Number of outputs:"; outputWidth "Output width [msb ... lsb]:"; outputBinaryPt "Output binary point position [msb ... lsb]:"; outputArithmeticType "Output arithmetic type (ufix=0, fix=1, bool=2) [msb ... lsb]:"; show_format "Print format string?"; outputToWorkspace "Output to workspace?"; variablePrefix "Variable name prefix:"; outputToModelAsWell "Output to model as well?"
      mask help:
      | Expands a 'bus' made using a bus_create or Xilinx
      | concat block.
      | The input will be divided into the specified number
      | of outputs with the specified arithmetic types.
      | Divisions are made from most significant bit.
      mask init: same as s_b16a4x512f/bus_expand
      settings: AttributesFormatString=2 outputs: uf16.0,uf48.0,
      mask TypeOptions mode: divisions of equal size | divisions of arbitrary size
      mask Callback mode: bus_expand_callback();
      mask Callback outputWidth: bus_expand_callback();
      mask Callback outputToWorkspace: bus_expand_callback();
  bus_expand7 : Subsystem  AncestorBlock=casper_library_flow_control/bus_expand  mask(bus_expand){mode=divisions of arbitrary size, outputNum=1, outputWidth=[16 48], outputBinaryPt=0, outputArithmeticType=0, show_format=on, outputToWorkspace=off, variablePrefix=out, outputToModelAsWell=on}
      mask prompts: outputNum "Number of outputs:"; outputWidth "Output width [msb ... lsb]:"; outputBinaryPt "Output binary point position [msb ... lsb]:"; outputArithmeticType "Output arithmetic type (ufix=0, fix=1, bool=2) [msb ... lsb]:"; show_format "Print format string?"; outputToWorkspace "Output to workspace?"; variablePrefix "Variable name prefix:"; outputToModelAsWell "Output to model as well?"
      mask help:
      | Expands a 'bus' made using a bus_create or Xilinx
      | concat block.
      | The input will be divided into the specified number
      | of outputs with the specified arithmetic types.
      | Divisions are made from most significant bit.
      mask init: same as s_b16a4x512f/bus_expand
      settings: AttributesFormatString=2 outputs: uf16.0,uf48.0,
      mask TypeOptions mode: divisions of equal size | divisions of arbitrary size
      mask Callback mode: bus_expand_callback();
      mask Callback outputWidth: bus_expand_callback();
      mask Callback outputToWorkspace: bus_expand_callback();
  bus_expand8 : Subsystem  AncestorBlock=casper_library_flow_control/bus_expand  mask(bus_expand){mode=divisions of arbitrary size, outputNum=1, outputWidth=[16 48], outputBinaryPt=0, outputArithmeticType=0, show_format=on, outputToWorkspace=off, variablePrefix=out, outputToModelAsWell=on}
      mask prompts: outputNum "Number of outputs:"; outputWidth "Output width [msb ... lsb]:"; outputBinaryPt "Output binary point position [msb ... lsb]:"; outputArithmeticType "Output arithmetic type (ufix=0, fix=1, bool=2) [msb ... lsb]:"; show_format "Print format string?"; outputToWorkspace "Output to workspace?"; variablePrefix "Variable name prefix:"; outputToModelAsWell "Output to model as well?"
      mask help:
      | Expands a 'bus' made using a bus_create or Xilinx
      | concat block.
      | The input will be divided into the specified number
      | of outputs with the specified arithmetic types.
      | Divisions are made from most significant bit.
      mask init: same as s_b16a4x512f/bus_expand
      settings: AttributesFormatString=2 outputs: uf16.0,uf48.0,
      mask TypeOptions mode: divisions of equal size | divisions of arbitrary size
      mask Callback mode: bus_expand_callback();
      mask Callback outputWidth: bus_expand_callback();
      mask Callback outputToWorkspace: bus_expand_callback();
  bus_expand9 : Subsystem  AncestorBlock=casper_library_flow_control/bus_expand  mask(bus_expand){mode=divisions of arbitrary size, outputNum=1, outputWidth=[16 48], outputBinaryPt=0, outputArithmeticType=0, show_format=on, outputToWorkspace=off, variablePrefix=out, outputToModelAsWell=on}
      mask prompts: outputNum "Number of outputs:"; outputWidth "Output width [msb ... lsb]:"; outputBinaryPt "Output binary point position [msb ... lsb]:"; outputArithmeticType "Output arithmetic type (ufix=0, fix=1, bool=2) [msb ... lsb]:"; show_format "Print format string?"; outputToWorkspace "Output to workspace?"; variablePrefix "Variable name prefix:"; outputToModelAsWell "Output to model as well?"
      mask help:
      | Expands a 'bus' made using a bus_create or Xilinx
      | concat block.
      | The input will be divided into the specified number
      | of outputs with the specified arithmetic types.
      | Divisions are made from most significant bit.
      mask init: same as s_b16a4x512f/bus_expand
      settings: AttributesFormatString=2 outputs: uf16.0,uf48.0,
      mask TypeOptions mode: divisions of equal size | divisions of arbitrary size
      mask Callback mode: bus_expand_callback();
      mask Callback outputWidth: bus_expand_callback();
      mask Callback outputToWorkspace: bus_expand_callback();
  edge_detect : Subsystem  AncestorBlock=casper_library_misc/edge_detect  mask(edge_detect){edge=Falling, polarity=Active High, x_in=[0 0.08 0.08 0.16 0.16 0.24 0.24 0.32 0.32 0.4], y_in=[-1 -1  1  1  1  1  1  1  1  1], x_out=[0.6 0.68 0.68 0.76 0.76 0.84 0.84 0.92 0.92 1], y_out=[-1 -1  1  1 -1 -1 -1 -1 -1 -1]}
      mask prompts: edge "Edge Type"; polarity "Output Polarity"; x_in "Input X Positions"; y_in "Input Y Positions"; x_out "Output X Positions"; y_out "Output Y Positions"
      mask help: Output is active for one-cycle after each edge of the specified type (i.e. rising, falling or both).
      mask init: same as s_b16a4x512f/edge_detect
      settings: AttributesFormatString=|
      | falling edges
      | active high
      mask Help: Output is active for one-cycle after each edge of the specified type (i.e. rising, falling, or both).  Latency is zero.
      mask TypeOptions edge: Rising | Falling | Both
      mask TypeOptions polarity: Active High | Active Low
      mask Display:
      | plot(x_in_num,0.5+y_in_num*0.2);
      | plot(x_out_num,0.5+y_out_num*0.2);
  header_4const11 : xbsIndex_r4/Constant  const=2  gui_display_data_type=Fixed-point  arith_type=Unsigned  n_bits=2  bin_pt=0  preci_type=Single  exp_width=8  frac_width=24  explicit_period=on  period=1  equ=P=C  opselect=C  inp2=PCIN>>17  opr=+  inp1=P  carry=CIN  dbl_ovrd=off  block_type=constant
  header_one : xbsIndex_r4/Concat  num_inputs=6  dbl_ovrd=off  block_type=concat
      settings: block_version=10.1.3
  header_reg{1,3..4,8} (4 alike) : xbsIndex_r4/Register  init=0  rst=off  en=on  dbl_ovrd=off  block_type=register
  heap_addr_width : xbsIndex_r4/Constant  const=spead_lsw/8  gui_display_data_type=Fixed-point  arith_type=Unsigned  n_bits=8  bin_pt=0  preci_type=Single  exp_width=8  frac_width=24  explicit_period=on  period=1  equ=P=C  opselect=C  inp2=PCIN>>17  opr=+  inp1=P  carry=CIN  dbl_ovrd=off  block_type=constant
  item_id_width : xbsIndex_r4/Constant  const=(spead_msw-spead_lsw)/8  gui_display_data_type=Fixed-point  arith_type=Unsigned  n_bits=8  bin_pt=0  preci_type=Single  exp_width=8  frac_width=24  explicit_period=on  period=1  equ=P=C  opselect=C  inp2=PCIN>>17  opr=+  inp1=P  carry=CIN  dbl_ovrd=off  block_type=constant
  num_item_pts : xbsIndex_r4/Constant  const=11  gui_display_data_type=Fixed-point  arith_type=Unsigned  n_bits=16  bin_pt=0  preci_type=Single  exp_width=8  frac_width=24  explicit_period=on  period=1  equ=P=C  opselect=C  inp2=PCIN>>17  opr=+  inp1=P  carry=CIN  dbl_ovrd=off  block_type=constant
  pkt_word_ctr : xbsIndex_r4/Counter  cnt_type=Free Running  cnt_to=Inf  operation=Up  start_count=0  cnt_by_val=1  arith_type=Unsigned  n_bits=max_pkt_len_bits-2  bin_pt=0  load_pin=off  rst=on  en=on  explicit_period=on  period=1  use_behavioral_HDL=off  implementation=Fabric  dbl_ovrd=off  block_type=counter
  pkt_start : Outport
  data256 : Outport  Port=2
  valid256 : Outport  Port=3
  eof256 : Outport  Port=4
  magic_error : Outport  Port=5
  hdr_error : Outport  Port=6
  pad_error : Outport  Port=7
  pkt_len_err : Outport  Port=8
  hdr_heap_id : Outport  Port=9
  hdr_heap_size : Outport  Port=10
  hdr_heap_offset : Outport  Port=11
  hdr_pkt_len : Outport  Port=12
  hdr5_0x1600_DIR : Outport  Port=13
  hdr6_0x4101_DIR : Outport  Port=14
  hdr7_0x4103_DIR : Outport  Port=15
  hdr8_0x4300 : Outport  Port=16
  tag scope: unpack_pkt_idx_g=global
  wires:
  pkt_valid/1 -> Assert7/1
  pkt_data/1 -> Assert5/1
  pkt_eof/1 -> Assert6/1
  Assert6/1 -> [gbe_eof]  "gbe_eof"
  Assert7/1 -> [gbe_valid]  "gbe_valid"
  Assert5/1 -> [gbe_data]  "gbe_data"
  num_item_pts/1 -> header_one/6
  Constant5/1 -> header_one/5
  heap_addr_width/1 -> header_one/4
  item_id_width/1 -> header_one/3
  Constant2/1 -> header_one/2
  Constant1/1 -> header_one/1
  header_one/1 -> Assert2/1  "hdr_exp"
  Assert2/1 -> [magic_word]
  Relational16/1 -> edge_detect/1(in), Logical/2, Logical8/2
  [gbe_valid] -> Logical/1  "gbe_valid"
  Logical/1 -> Scope3/3, [hdr_en]  "hdr_busy"
  header_reg3/1 -> Scope1/3, [hdr_1], header_reg4/1
  header_reg4/1 -> Scope1/2, [hdr_0]
  [hdr_1] -> bus_expand/1(bus_in)
  bus_expand/1(msb_out4) -> bus_expand1/1(bus_in)
  bus_expand/2(out3) -> bus_expand2/1(bus_in)
  bus_expand/3(out2) -> bus_expand3/1(bus_in)
  bus_expand/4(lsb_out1) -> bus_expand4/1(bus_in)
  bus_expand1/1(msb_out2) -> Relational4/2  "id0"
  bus_expand3/2(lsb_out1) -> [hdr_4101]  "val2"
  bus_expand4/2(lsb_out1) -> [hdr_4103]  "val3"
  bus_expand4/1(msb_out2) -> Relational7/2  "id3"
  bus_expand3/1(msb_out2) -> Relational6/2  "id2"
  bus_expand2/1(msb_out2) -> Relational5/2  "id1"
  bus_expand2/2(lsb_out1) -> [hdr_1600]  "val1"
  bus_expand1/2(lsb_out1) -> [pkt_len_bytes]  "val0"
  header_reg1/1 -> Scope1/4, [hdr_2], header_reg3/1
  [gbe_data] -> header_reg1/1
  [hdr_en] -> header_reg3/2, Scope1/1, header_reg4/2, header_reg1/2
  [hdr_2] -> bus_expand5/1(bus_in)
  bus_expand5/1(msb_out4) -> bus_expand6/1(bus_in)
  bus_expand5/2(out3) -> bus_expand7/1(bus_in)
  bus_expand5/3(out2) -> bus_expand8/1(bus_in)
  bus_expand5/4(lsb_out1) -> bus_expand9/1(bus_in)
  bus_expand6/1(msb_out2) -> Relational8/2  "id0"
  bus_expand7/1(msb_out2) -> Relational9/2  "id1"
  bus_expand7/2(lsb_out1) -> Relational10/2  "val1"
  bus_expand6/2(lsb_out1) -> [hdr_4300]  "val0"
  bus_expand10/1(msb_out4) -> Relational/2, bus_expand15/1(bus_in)  "w3"
  bus_expand10/2(out3) -> bus_expand12/1(bus_in)  "w2"
  bus_expand10/3(out2) -> bus_expand13/1(bus_in)  "w1"
  bus_expand10/4(lsb_out1) -> bus_expand14/1(bus_in)  "w0"
  bus_expand13/2(lsb_out1) -> [heap_size]  "val2"
  bus_expand14/2(lsb_out1) -> [heap_offset]  "val3"
  bus_expand14/1(msb_out2) -> Relational3/2  "id3"
  bus_expand13/1(msb_out2) -> Relational2/2  "id2"
  bus_expand12/1(msb_out2) -> Relational1/2  "id1"
  bus_expand12/2(lsb_out1) -> [heap_id]  "val1"
  bus_expand15/1(msb_out6) -> Terminator26/1  "magic0"
  bus_expand15/2(out5) -> Terminator27/1  "magic1"
  bus_expand15/3(out4) -> Terminator24/1  "magic2"
  bus_expand15/4(out3) -> Terminator25/1  "magic3"
  bus_expand15/5(out2) -> Terminator16/1  "magic4"
  bus_expand15/6(lsb_out1) -> Terminator17/1  "magic5"
  [magic_word] -> Relational/1
  [heap_id] -> Delay8/1  "heap_id"
  [heap_size] -> Delay7/1  "heap_size"
  [heap_offset] -> Delay6/1  "heap_offset"
  [pkt_len_bytes] -> Delay5/1  "pkt_len"
  [hdr_1600] -> Delay4/1  "0x1600"
  [hdr_4101] -> Delay3/1  "0x4101"
  [hdr_4103] -> Delay2/1  "0x4103"
  [hdr_4300] -> Delay1/1  "0x4300"
  edge_detect/1(out) -> Scope3/4, [pkt_start]  "pkt_start"
  [pkt_start] -> Delay12/1  "pkt_start"
  Relational/1 -> [error0]  "magic_error"
  Relational1/1 -> [error1]
  Constant/1 -> Relational1/1
  Relational2/1 -> [error2]
  Constant3/1 -> Relational2/1
  Relational3/1 -> [error3]
  Constant4/1 -> Relational3/1
  Relational4/1 -> [error4]
  Constant6/1 -> Relational4/1
  Relational5/1 -> [error5]
  Constant7/1 -> Relational5/1
  Relational6/1 -> [error6]
  Constant8/1 -> Relational6/1
  Relational7/1 -> [error7]
  Constant9/1 -> Relational7/1
  Relational8/1 -> [error8]
  Constant10/1 -> Relational8/1
  Relational9/1 -> [error9]
  Constant11/1 -> Relational9/1
  Relational10/1 -> [pad_error_0]
  Constant12/1 -> Relational10/1
  bus_expand8/1(msb_out2) -> Relational12/2  "id2"
  bus_expand8/2(lsb_out1) -> Relational11/2  "val2"
  Relational12/1 -> [error10]
  Constant13/1 -> Relational12/1
  Relational11/1 -> [pad_error_1]
  Constant14/1 -> Relational11/1
  Relational14/1 -> [error11]
  Constant15/1 -> Relational14/1
  Relational13/1 -> [pad_error_2]
  Constant16/1 -> Relational13/1
  bus_expand9/1(msb_out2) -> Relational14/2  "id3"
  bus_expand9/2(lsb_out1) -> Relational13/2  "val3"
  [pad_error_1] -> Logical1/2
  [pad_error_0] -> Logical1/1
  [pad_error_2] -> Logical1/3
  [error1] -> Logical2/1
  [error10] -> Logical2/10
  [error6] -> Logical2/6
  [error8] -> Logical2/8
  [error2] -> Logical2/2
  [error5] -> Logical2/5
  [error7] -> Logical2/7
  [error3] -> Logical2/3
  [error9] -> Logical2/9
  [error11] -> Logical2/11
  [error4] -> Logical2/4
  [error0] -> Logical3/2
  [pkt_start] -> Logical3/1
  [pkt_start] -> Logical4/1
  [pkt_start] -> Logical5/1
  Logical2/1 -> Logical5/2
  Logical1/1 -> Logical4/2
  Logical3/1 -> [error_magic]  "error_magic"
  Logical4/1 -> [error_pad]  "error_pad"
  Logical5/1 -> [error_hdr]  "error_hdr"
  [error_magic] -> magic_error/1
  [hdr_en] -> Inverter/1
  Delay10/1 -> Logical6/1
  [gbe_data] -> Delay11/1  "data256"
  Logical6/1 -> valid256/1  "valid256"
  [gbe_eof] -> Delay9/1  "eof256"
  [hdr_en] -> Scope2/4, pkt_word_ctr/1
  [gbe_valid] -> pkt_word_ctr/2
  pkt_word_ctr/1 -> Slice1/1, Scope2/1, Relational15/2  "pkt_ctr"
  [pkt_len_bytes] -> Slice/1
  Slice/1 -> Delay15/1  "pkt_len_from_hdr"
  Relational15/1 -> Logical9/1
  [gbe_eof] -> Scope2/3, Delay/1
  Logical9/1 -> [error_pkt_len]  "pkt_len_err"
  Delay/1 -> Logical9/2
  [error_pkt_len] -> pkt_len_err/1
  [hdr_0] -> bus_expand10/1(bus_in)
  [error_pad] -> pad_error/1
  [error_hdr] -> hdr_error/1
  [error_pad] -> Logical7/3
  [error_magic] -> Logical7/1
  [error_hdr] -> Logical7/2
  Logical7/1 -> Inverter1/1
  [pkt_start] -> header_reg8/2
  header_reg8/1 -> Logical6/3
  Delay1/1 -> hdr8_0x4300/1
  Delay2/1 -> hdr7_0x4103_DIR/1
  Delay3/1 -> hdr6_0x4101_DIR/1
  Delay4/1 -> hdr5_0x1600_DIR/1
  Delay5/1 -> hdr_pkt_len/1
  Delay6/1 -> hdr_heap_offset/1
  Delay7/1 -> hdr_heap_size/1
  Delay8/1 -> hdr_heap_id/1
  Delay9/1 -> eof256/1
  Delay11/1 -> data256/1
  Delay12/1 -> pkt_start/1
  Delay13/1 -> Logical6/2
  [gbe_valid] -> Delay13/1
  Inverter/1 -> Delay10/1
  Inverter1/1 -> header_reg8/1
  header_4const11/1 -> Relational16/2
  Counter1/1 -> Relational16/1
  Logical8/1 -> Counter1/2
  [gbe_eof] -> Counter1/1
  [gbe_valid] -> Logical8/1
  [gbe_eof] -> Scope3/1
  [gbe_valid] -> Scope3/2
  [hdr_en] -> Mux/1
  Mux/1 -> Scope2/2
  [gbe_data] -> Mux/2
  Constant17/1 -> Mux/3
  Delay15/1 -> Relational15/1
  Slice1/1 -> [unpack_pkt_idx_g]
